simulink model "PIDGuideOnLoadDiscrete"  (R2016a)
settings: Solver=VariableStepAuto  StartTime=0.0  StopTime=10.0  RelTol=1e-3
undefined symbols (not defined in the file or in its folder): DLeftWS, DRightWS, ILeftWS, IRightWS, NLeftWS, NRightWS, PLeftWS, PRightWS
libraries: simulink x2
settings Model: Creator=kkhan  LastModifiedBy=kkhan

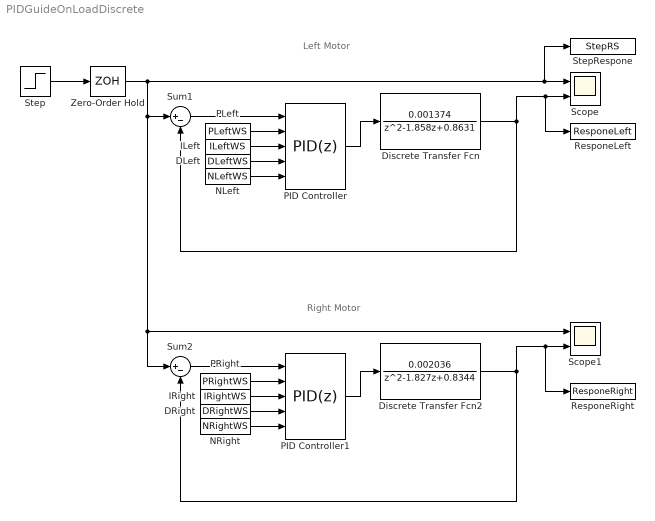
== system PIDGuideOnLoadDiscrete ==
  note: Right Motor
  note: Left Motor
  DLeft : Constant  Value=DLeftWS  SampleTime=0.02
  DRight : Constant  Value=DRightWS  SampleTime=0.02
  Discrete Transfer Fcn : DiscreteTransferFcn  Numerator=[0.001374]  Denominator=[1 -1.858 0.8631]  SampleTime=0.02
  Discrete Transfer Fcn2 : DiscreteTransferFcn  Numerator=[0.002036]  Denominator=[1 -1.827 0.8344]  SampleTime=0.02
  "ILeft " : Constant  Value=ILeftWS  SampleTime=0.02
  IRight : Constant  Value=IRightWS  SampleTime=0.02
  NLeft : Constant  Value=NLeftWS  SampleTime=0.02
  NRight : Constant  Value=NRightWS  SampleTime=0.02
  PID Controller : simulink/Continuous/PID Controller  Controller=PID  TimeDomain=Discrete-time  SampleTime=0.02  IntegratorMethod=Forward Euler  FilterMethod=Forward Euler  Form=Parallel  UseFilter=on  ControllerParametersSource=external  P=21.0909852919714  I=43.5478218388463  D=2.15960697462874  N=26.7883535297543  InitialConditionSource=internal  InitialConditionForIntegrator=0  InitialConditionForFilter=0  ExternalReset=none  LimitOutput=off  UpperSaturationLimit=inf  LowerSaturationLimit=-inf  LinearizeAsGain=on  AntiWindupMode=none  Kb=1  TrackingMode=off  Kt=1  PParamMin=[]  PParamMax=[]  IParamMin=[]  IParamMax=[]  DParamMin=[]  DParamMax=[]  NParamMin=[]  NParamMax=[]  KbParamMin=[]  KbParamMax=[]  KtParamMin=[]  KtParamMax=[]  POutMin=[]  POutMax=[]  IOutMin=[]  IOutMax=[]  DOutMin=[]  DOutMax=[]  NOutMin=[]  NOutMax=[]  KbOutMin=[]  KbOutMax=[]  KtOutMin=[]  KtOutMax=[]  IntegratorOutMin=[]  IntegratorOutMax=[]  FilterOutMin=[]  FilterOutMax=[]  SumOutMin=[]  SumOutMax=[]  SumI1OutMin=[]  SumI1OutMax=[]  SumI2OutMin=[]  SumI2OutMax=[]  SumI3OutMin=[]  SumI3OutMax=[]  SumDOutMin=[]  SumDOutMax=[]  SaturationOutMin=[]  SaturationOutMax=[]  IntegratorContinuousStateAttributes=''  IntegratorStateMustResolveToSignalObject=off  IntegratorRTWStateStorageClass=Auto  FilterContinuousStateAttributes=''  FilterStateMustResolveToSignalObject=off  FilterRTWStateStorageClass=Auto  DifferentiatorICPrevScaledInput=0  DifferentiatorOutMin=[]  DifferentiatorOutMax=[]
  PID Controller1 : simulink/Continuous/PID Controller  Controller=PID  TimeDomain=Discrete-time  SampleTime=0.02  IntegratorMethod=Forward Euler  FilterMethod=Forward Euler  Form=Parallel  UseFilter=on  ControllerParametersSource=external  P=21.0909852919714  I=43.5478218388463  D=2.15960697462874  N=26.7883535297543  InitialConditionSource=internal  InitialConditionForIntegrator=0  InitialConditionForFilter=0  ExternalReset=none  LimitOutput=off  UpperSaturationLimit=inf  LowerSaturationLimit=-inf  LinearizeAsGain=on  AntiWindupMode=none  Kb=1  TrackingMode=off  Kt=1  PParamMin=[]  PParamMax=[]  IParamMin=[]  IParamMax=[]  DParamMin=[]  DParamMax=[]  NParamMin=[]  NParamMax=[]  KbParamMin=[]  KbParamMax=[]  KtParamMin=[]  KtParamMax=[]  POutMin=[]  POutMax=[]  IOutMin=[]  IOutMax=[]  DOutMin=[]  DOutMax=[]  NOutMin=[]  NOutMax=[]  KbOutMin=[]  KbOutMax=[]  KtOutMin=[]  KtOutMax=[]  IntegratorOutMin=[]  IntegratorOutMax=[]  FilterOutMin=[]  FilterOutMax=[]  SumOutMin=[]  SumOutMax=[]  SumI1OutMin=[]  SumI1OutMax=[]  SumI2OutMin=[]  SumI2OutMax=[]  SumI3OutMin=[]  SumI3OutMax=[]  SumDOutMin=[]  SumDOutMax=[]  SaturationOutMin=[]  SaturationOutMax=[]  IntegratorContinuousStateAttributes=''  IntegratorStateMustResolveToSignalObject=off  IntegratorRTWStateStorageClass=Auto  FilterContinuousStateAttributes=''  FilterStateMustResolveToSignalObject=off  FilterRTWStateStorageClass=Auto  DifferentiatorICPrevScaledInput=0  DifferentiatorOutMin=[]  DifferentiatorOutMax=[]
  "PLeft " : Constant  Value=PLeftWS  SampleTime=0.02
  PRight : Constant  Value=PRightWS  SampleTime=0.02
  ResponeLeft : ToWorkspace  VariableName=ResponeLeft  SaveFormat=Timeseries  SampleTime=0.02
  ResponeRight : ToWorkspace  VariableName=ResponeRight  SaveFormat=Timeseries  SampleTime=0.02
  Scope : Scope  NumInputPorts=2
  Scope1 : Scope  NumInputPorts=2
  Step : Step  Time=0  After=50
  StepRespone : ToWorkspace  VariableName=StepRS  SaveFormat=Timeseries  SampleTime=0.02
  Sum1 : Sum  Inputs=|+-
  Sum2 : Sum  Inputs=|+-
  Zero-Order Hold : ZeroOrderHold  SampleTime=0.02
  wires:
  Step/1 -> Zero-Order Hold/1
  Sum1/1 -> PID Controller/1
  Discrete Transfer Fcn/1 -> Sum1/2, ResponeLeft/1, Scope/2
  PID Controller/1 -> Discrete Transfer Fcn/1
  "PLeft "/1 -> PID Controller/2
  Sum2/1 -> PID Controller1/1
  Discrete Transfer Fcn2/1 -> Sum2/2, ResponeRight/1, Scope1/2
  PID Controller1/1 -> Discrete Transfer Fcn2/1
  Zero-Order Hold/1 -> StepRespone/1, Scope/1, Scope1/1, Sum2/1, Sum1/1
  "ILeft "/1 -> PID Controller/3
  DLeft/1 -> PID Controller/4
  NLeft/1 -> PID Controller/5
  PRight/1 -> PID Controller1/2
  IRight/1 -> PID Controller1/3
  DRight/1 -> PID Controller1/4
  NRight/1 -> PID Controller1/5
